simulink model "LabPSU_CPU02"  (R2026b)
undefined symbols (not defined in the file or in its folder): Com_ipcTs
libraries: c280xlib x2, procinterlib x2, c2000lib x1, c2837xDlib x1
settings Model: Creator=BenjaminRupp  LastModifiedBy=BenjaminRupp

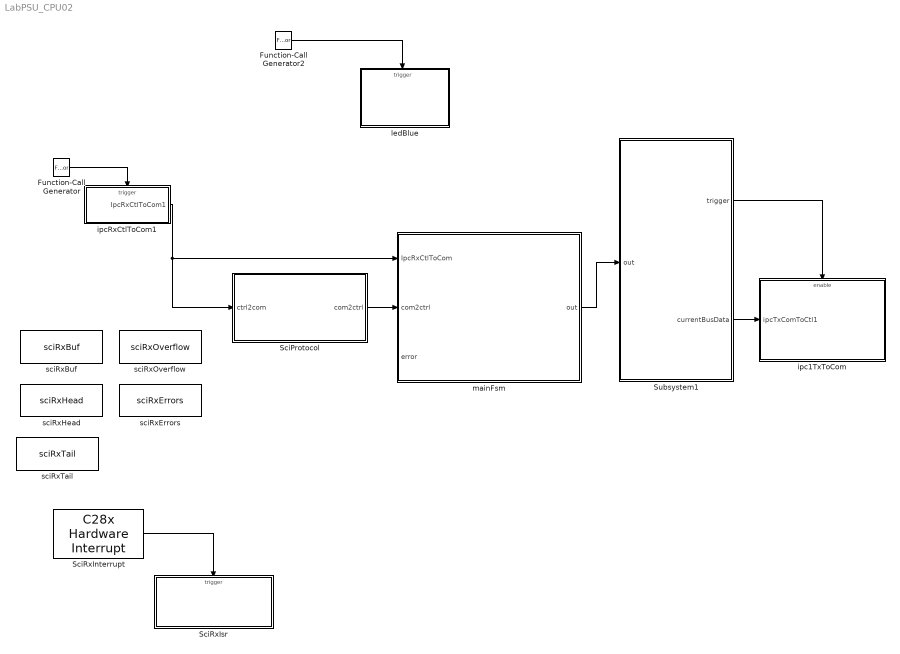
== system LabPSU_CPU02 ==
  Function-Call Generator : FunctionCallGenerator  SampleTime=Com_ipcTs
  Function-Call Generator2 : FunctionCallGenerator  SampleTime=0.1
  SciProtocol : Subsystem  TreatAsAtomicUnit=on  SystemSampleTime=Com_ipcTs
  SciRxInterrupt : c2000lib/Scheduling/C28x Hardware Interrupt  irqnumbers=[9]  pienumbers=[1]  irqpriorities=[30]  irqpreempts=0  showinput=off  dspchiptype=C280X
  SciRxIsr : Subsystem
  Subsystem1 : Subsystem
  ipc1TxToCom : Subsystem
  ipcRxCtlToCom1 : Subsystem
  ledBlue : Subsystem
  mainFsm : Subsystem
  sciRxBuf : DataStoreMemory  DataStoreName=sciRxBuf  InitialValue=zeros(64,1)  ShowAdditionalParam=off  OutDataTypeStr=uint16
  sciRxErrors : DataStoreMemory  DataStoreName=sciRxErrors  ShowAdditionalParam=off  OutDataTypeStr=uint16
  sciRxHead : DataStoreMemory  DataStoreName=sciRxHead  ShowAdditionalParam=off  OutDataTypeStr=uint16
  sciRxOverflow : DataStoreMemory  DataStoreName=sciRxOverflow  ShowAdditionalParam=off  OutDataTypeStr=uint16
  sciRxTail : DataStoreMemory  DataStoreName=sciRxTail  ShowAdditionalParam=off  OutDataTypeStr=uint16
  wires:
  Function-Call Generator/1 -> ipcRxCtlToCom1/Trigger
  ipcRxCtlToCom1/1(IpcRxCtlToCom1) -> SciProtocol/1(ctrl2com), mainFsm/1(IpcRxCtlToCom)
  Function-Call Generator2/1 -> ledBlue/Trigger
  mainFsm/1(out) -> Subsystem1/1(out)
  Subsystem1/2(currentBusData) -> ipc1TxToCom/1(ipcTxComToCtl1)
  Subsystem1/1(trigger) -> ipc1TxToCom/Enable
  SciProtocol/1(com2ctrl) -> mainFsm/2(com2ctrl)
  SciRxInterrupt/1 -> SciRxIsr/Trigger

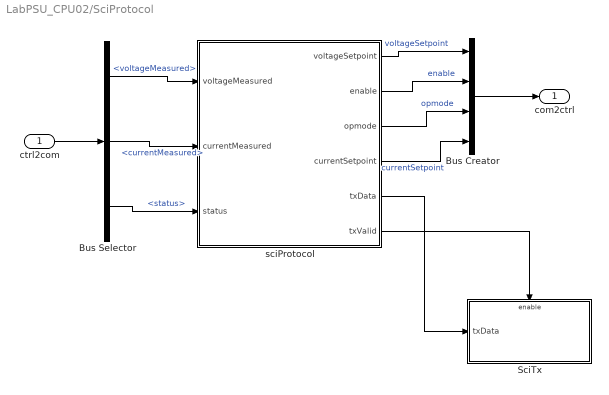
== system LabPSU_CPU02/SciProtocol ==
  ctrl2com : Inport  OutDataTypeStr=Bus: ctrl2com
  Bus Creator : BusCreator  Inputs=4  OutDataTypeStr=Bus: com2ctrl
  Bus Selector : BusSelector  OutputSignals=voltageMeasured,currentMeasured,status
  SciTx : Subsystem
  sciProtocol : MATLAB Function  TreatAsAtomicUnit=on
  com2ctrl : Outport  OutDataTypeStr=Bus: com2ctrl
  wires:
  sciProtocol/6(txValid) -> SciTx/Enable
  sciProtocol/5(txData) -> SciTx/1(txData)
  Bus Creator/1 -> com2ctrl/1
  sciProtocol/4(currentSetpoint) -> Bus Creator/4  "currentSetpoint"
  sciProtocol/3(opmode) -> Bus Creator/3  "opmode"
  sciProtocol/2(enable) -> Bus Creator/2  "enable"
  sciProtocol/1(voltageSetpoint) -> Bus Creator/1  "voltageSetpoint"
  Bus Selector/3 -> sciProtocol/3(status)  "<status>"
  Bus Selector/2 -> sciProtocol/2(currentMeasured)  "<currentMeasured>"
  Bus Selector/1 -> sciProtocol/1(voltageMeasured)  "<voltageMeasured>"
  ctrl2com/1 -> Bus Selector/1

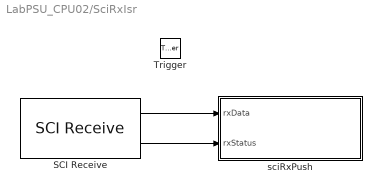
== system LabPSU_CPU02/SciRxIsr ==
  Trigger : TriggerPort  TriggerType=function-call  VariantControl=(inherit)
  SCI Receive : c280xlib/SCI Receive  Priority=2  sciModule=A  dataHead=''  headerCheckMaxCount=16  dataTail=''  dataType=uint8  dataLenOptions=Length via dialog  dataDim=1  maxDataLength=1  initValue=0  errOption=Output the last received value  errValue=0  sampleTime=-1  blockingMode=off  timeOut=inf  outputStatus=on
      settings: LibrarySourceBlock=c2837xDlib/SCI Receive
  sciRxPush : MATLAB Function  TreatAsAtomicUnit=on
  wires:
  SCI Receive/2 -> sciRxPush/2(rxStatus)
  SCI Receive/1 -> sciRxPush/1(rxData)

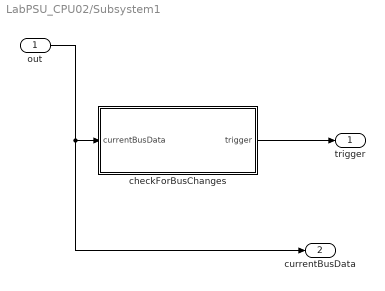
== system LabPSU_CPU02/Subsystem1 ==
  out : Inport
  checkForBusChanges : MATLAB Function  TreatAsAtomicUnit=on
  trigger : Outport
  currentBusData : Outport  Port=2
  wires:
  checkForBusChanges/1(trigger) -> trigger/1
  out/1 -> checkForBusChanges/1(currentBusData), currentBusData/1

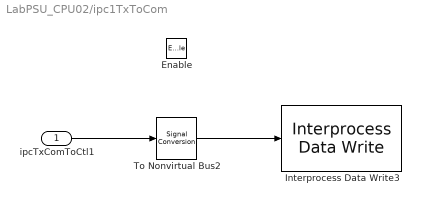
== system LabPSU_CPU02/ipc1TxToCom ==
  ipcTxComToCtl1 : Inport  OutDataTypeStr=Bus: com2ctrl
  Enable : EnablePort
  Interprocess Data Write3 : procinterlib/Interprocess Data Write  Priority=3  showPort=off  ChannelNum=1  NumBuff=1  IsIntEnabled=1  EnInterrupt=on  IPCBetween=0  CurrentPU=1  DataType=uint8  PartCores=CPU1<->CPU2  TargetType=0  ClientPU=TriCore1  ClientIntPrio=50  CurrentPUPriority=0  TargetName=0
      settings: LibrarySourceBlock=c2000lib/Target Communication/Interprocess Data Write
  To Nonvirtual Bus2 : SignalConversion  ConversionOutput=Nonvirtual bus  OverrideOpt=off
  wires:
  ipcTxComToCtl1/1 -> To Nonvirtual Bus2/1
  To Nonvirtual Bus2/1 -> Interprocess Data Write3/1

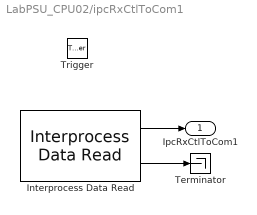
== system LabPSU_CPU02/ipcRxCtlToCom1 ==
  Trigger : TriggerPort  TriggerType=function-call  VariantControl=(inherit)  PortDimensions=1
  Interprocess Data Read : procinterlib/Interprocess Data Read  showPort=off  DataType=Bus: ctrl2com  NumBuffers=1  DataLength=1  ChannelNum=6  IsIntEnabled=0  EnInterrupt=off  StructForBus=struct('voltageMeasured',single(zeros(1,1)),'currentMeasured',single(zeros(1,1)),'status',uint16(zeros(1,1)))  IPCBetween=0  CurrentPU=1  PartCores=CPU1<->CPU2  SampleTime=-1  TargetType=0  ClientPU=TriCore1  ClientIntPrio=50  CurrentPUPriority=0  TargetName=0
      settings: LibrarySourceBlock=c2000lib/Target Communication/Interprocess Data Read
  Terminator : Terminator
  IpcRxCtlToCom1 : Outport  OutDataTypeStr=Bus: ctrl2com
  wires:
  Interprocess Data Read/2 -> Terminator/1
  Interprocess Data Read/1 -> IpcRxCtlToCom1/1

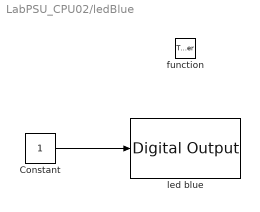
== system LabPSU_CPU02/ledBlue ==
  function : TriggerPort  TriggerType=function-call  VariantControl=(inherit)
  Constant : Constant
  led blue : c2837xDlib/Digital Output  GPIO_Number=GPIO32~GPIO39  GPIO_Bit0=off  GPIO_BIT0_Toggle=off  GPIO_Bit1=off  GPIO_BIT1_Toggle=off  GPIO_Bit2=on  GPIO_BIT2_Toggle=on  GPIO_Bit3=off  GPIO_BIT3_Toggle=off  GPIO_Bit4=off  GPIO_BIT4_Toggle=off  GPIO_Bit5=off  GPIO_BIT5_Toggle=off  GPIO_Bit6=off  GPIO_BIT6_Toggle=off  GPIO_Bit7=off  GPIO_BIT7_Toggle=off
  wires:
  Constant/1 -> led blue/1

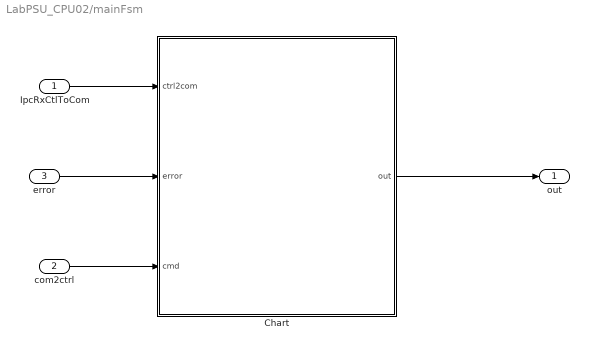
== system LabPSU_CPU02/mainFsm ==
  IpcRxCtlToCom : Inport  OutDataTypeStr=Bus: ctrl2com
  com2ctrl : Inport  Port=2  OutDataTypeStr=Bus: com2ctrl
  error : Inport  Port=3
  Chart : Stateflow chart  TreatAsAtomicUnit=on
  out : Outport  OutDataTypeStr=Bus: com2ctrl
  wires:
  error/1 -> Chart/2(error)
  Chart/1(out) -> out/1
  com2ctrl/1 -> Chart/3(cmd)
  IpcRxCtlToCom/1 -> Chart/1(ctrl2com)

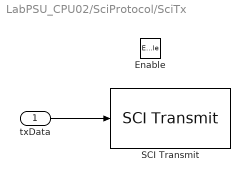
== system LabPSU_CPU02/SciProtocol/SciTx ==
  txData : Inport
  Enable : EnablePort
  SCI Transmit : c280xlib/SCI Transmit  sciModule=A  dataHead=''  dataTail=''  frameSize=1  blockingMode=on  outputStatus=off
      settings: LibrarySourceBlock=c2837xDlib/SCI Transmit
  wires:
  txData/1 -> SCI Transmit/1

== matlab function LabPSU_CPU02/SciRxIsr/sciRxPush ==
  data: rxData input; rxStatus input; sciRxBuf data_store_memory; sciRxHead data_store_memory; sciRxTail data_store_memory; sciRxOverflow data_store_memory; sciRxErrors data_store_memory
function sciRxPush(rxData, rxStatus)
%#codegen
% Runs in the SCI RX interrupt. Appends the received bytes to the ring
% buffer sciRxBuf. Only this function writes sciRxHead (single producer).
global sciRxBuf sciRxHead sciRxTail sciRxOverflow sciRxErrors  % Data Store Memory
mask = uint16(63);
if rxStatus ~= 0
    sciRxErrors = sciRxErrors + uint16(1);
    return;
end
for k = 1:numel(rxData)
    next = bitand(sciRxHead + uint16(1), mask);
    if next == sciRxTail
        sciRxOverflow = sciRxOverflow + uint16(1);
    else
        % No 8-bit type on C28x: store each byte in a uint16
        sciRxBuf(sciRxHead + 1) = bitand(uint16(rxData(k)), uint16(255));
        sciRxHead = next;
    end
end

== matlab function LabPSU_CPU02/Subsystem1/checkForBusChanges ==
  data: currentBusData input; trigger output boolean
function trigger = checkForBusChanges(currentBusData)
%% checkForBusChanges
% attach any Simulink Bus as input (can also be nested busses)
% if any of the elements in any of the leave bus has changed since the last
% call, the trigger is se to true, otherwise it's false.

persistent oldBusData;
if isempty(oldBusData)
    oldBusData = currentBusData;
    trigger = false;
    return
end


 % Compare current bus with previous bus recursively
    trigger = hasChanged(currentBusData, oldBusData);

    % Update previous bus with the current values
    oldBusData = currentBusData;
end


%% hasChanged 

function flag = hasChanged(curr, prev)
    % Recursively check if any element in the nested struct has changed
    flag = false;

    fields = fieldnames(curr);
    for i = 1:numel(fields)
        field = fields{i};
        
        if isstruct(curr.(field)) 
            % Recursively check nested structs (sub-buses)
            if hasChanged(curr.(field), prev.(field))
                flag = true;
                return;
            end
        else
            % Compare primitive values
            if ~isequal(curr.(field), prev.(field))
                flag = true;
                return;
            end
        end
    end
end

== matlab function LabPSU_CPU02/SciProtocol/sciProtocol ==
  data: voltageMeasured input; voltageSetpoint output single size=1; currentMeasured input; status input; enable output uint16 size=1; opmode output uint16 size=1; currentSetpoint output single size=1; txData output uint8 size=[12 1]; txValid output boolean size=1; sciRxBuf data_store_memory; sciRxHead data_store_memory; sciRxTail data_store_memory
function [voltageSetpoint, enable, opmode, currentSetpoint, txData, txValid] = ...
    sciProtocol(voltageMeasured, currentMeasured, status)
%#codegen
% SCI protocol, see docs/sci_protocol.md.
% Frame (12 bytes, little-endian): A5 5A | cmd(2) | key(2) | value(4) | 5A A5
% Runs at Com_ipcTs. Pops bytes from the ring buffer into a sliding
% 12-byte window and answers at most one frame per call (the 12-byte
% response fits into the 16-byte SCI TX FIFO). Only this function
% writes sciRxTail (single consumer).

global sciRxBuf sciRxHead sciRxTail  % Data Store Memory
persistent win vSet iSet en om started
if isempty(win)
    win = zeros(12, 1, 'uint16');
    vSet = single(0);
    iSet = single(0);
    en = uint16(0);
    om = uint16(0);
    started = false;
end

mask = uint16(63);

% Send the defaults to CPU1 once after reset.
started = true;
txData = zeros(12, 1, 'uint8');
txValid = false;

% Snapshot of the head: bytes received after this are handled next call.
head = sciRxHead;
while sciRxTail ~= head && ~txValid
    b = sciRxBuf(sciRxTail + 1);
    sciRxTail = bitand(sciRxTail + uint16(1), mask);
    win(1:11) = win(2:12);
    win(12) = b;

    if win(1) == 0xA5u16 && win(2) == 0x5Au16 && win(11) == 0x5Au16 && win(12) == 0xA5u16
        cmd   = bitor(uint16(win(3)), bitshift(uint16(win(4)), 8));
        key   = bitor(uint16(win(5)), bitshift(uint16(win(6)), 8));
        value = bitor(bitor(uint32(win(7)), bitshift(uint32(win(8)), 8)), ...
                      bitor(bitshift(uint32(win(9)), 16), bitshift(uint32(win(10)), 24)));

        err = uint32(0);
        respCmd = uint16(0);
        respValue = uint32(0);

        if cmd == 0x0001u16  % READ
            respCmd = 0x8001u16;
            switch key
                case 0x0001u16, respValue = typecast(vSet, 'uint32');
                case 0x0002u16, respValue = typecast(iSet, 'uint32');
                case 0x0003u16, respValue = uint32(en);
                case 0x0004u16, respValue = uint32(om);
                case 0x0101u16, respValue = typecast(single(voltageMeasured), 'uint32');
                case 0x0102u16, respValue = typecast(single(currentMeasured), 'uint32');
                case 0x0103u16, respValue = uint32(status);
                otherwise,   err = uint32(2);  % unknown key
            end
        elseif cmd == 0x0002u16  % WRITE
            respCmd = 0x8002u16;
            respValue = value;
            f = typecast(value, 'single');
            switch key
                case 0x0001u16
                    if isfinite(f) && f >= 0
                        vSet = f;
                    else
                        err = uint32(4);
                    end
                case 0x0002u16
                    if isfinite(f) && f >= 0
                        iSet = f;
                    else
                        err = uint32(4);
                    end
                case 0x0003u16  % 0 = off, 1 = on
                    if value <= 1
                        en = uint16(value);
                    else
                        err = uint32(4);
                    end
                case 0x0004u16  % 1 = closed loop, 2 = open loop, 3 = reserved, others don't care
                    if value <= 65535
                        om = uint16(value);
                    else
                        err = uint32(4);
                    end
                case {0x0101u16, 0x0102u16, 0x0103u16}
                    err = uint32(3);  % read-only
                otherwise
                    err = uint32(2);  % unknown key
            end
        else
            err = uint32(1);  % unknown command
        end

        if err ~= 0
            respCmd = 0x80FFu16;
            respValue = err;
        end

        txData(1)  = uint8(0xA5);
        txData(2)  = uint8(0x5A);
        txData(3)  = uint8(bitand(respCmd, uint16(255)));
        txData(4)  = uint8(bitshift(respCmd, -8));
        txData(5)  = uint8(bitand(key, uint16(255)));
        txData(6)  = uint8(bitshift(key, -8));
        for k = 0:3
            txData(7 + k) = uint8(bitand(bitshift(respValue, -8 * k), uint32(255)));
        end
        txData(11) = uint8(0x5A);
        txData(12) = uint8(0xA5);
        txValid = true;
        win(:) = 0;
    end
end

voltageSetpoint = vSet;
enable = en;
opmode = om;
currentSetpoint = iSet;

== stateflow chart LabPSU_CPU02/mainFsm/Chart ==
  state init
    en:
    out.currentSetpoint = single(0);
    out.enable = uint16(0);
    out.opmode = uint16(2);
    out.voltageSetpoint = single(0);
  state Operation
    en:
    out.enable = uint16(1);
    state openLoop
      en:
      out.opmode = uint16(2);
      du:
      out.voltageSetpoint = single(0);
      out.currentSetpoint = cmd.currentSetpoint;
    state closedLoop
      en:
      out.opmode = uint16(1);
      state ramping
        en, du:
        out.voltageSetpoint = cmd.voltageSetpoint;
      state atSetpoint
      (default) -> ramping
      atSetpoint -> ramping : [out.voltageSetpoint ~= cmd.voltageSetpoint]
      ramping -> atSetpoint : [abs(ctrl2com.voltageMeasured-cmd.voltageSetpoint)<voltageResolution]
    (default) -> closedLoop
    closedLoop -> openLoop : [cmd.opmode == uint16(2)]
  state Error
    en:
    out.currentSetpoint = single(0);
    out.enable = uint16(0);
    out.opmode = uint16(2);
    out.voltageSetpoint = single(0);
  (default) -> init
  Error -> init : [~error && ~cmd.enable]
  init -> Operation : [cmd.enable]
  Operation -> init [order 2] : [~cmd.enable]
  Operation -> Error [order 1] : [error]
  data: ctrl2com input; error input; cmd input; out output Bus: com2ctrl; voltageResolution constant single =1
